simulink model "FM_Stereo_System"  (R2025b)
settings: Solver=FixedStepAuto  StartTime=0.0  StopTime=0.05  FixedStep=Ts  RelTol=1e-3
values from neighbouring files (symbols this model uses):
  Ts = 3e-7    (= 3e-07)    [run_simulink_figures.m]
libraries: dspfdesign x8, commanapbnd3 x2
settings Model: Creator=alfre  LastModifiedBy=alfre

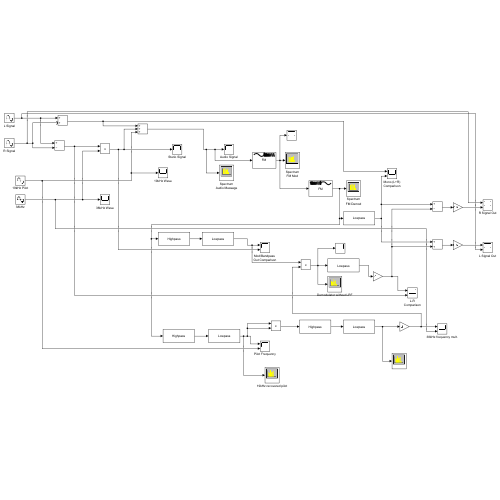
[thumbnail: Simulink's stored preview of the top-level diagram]
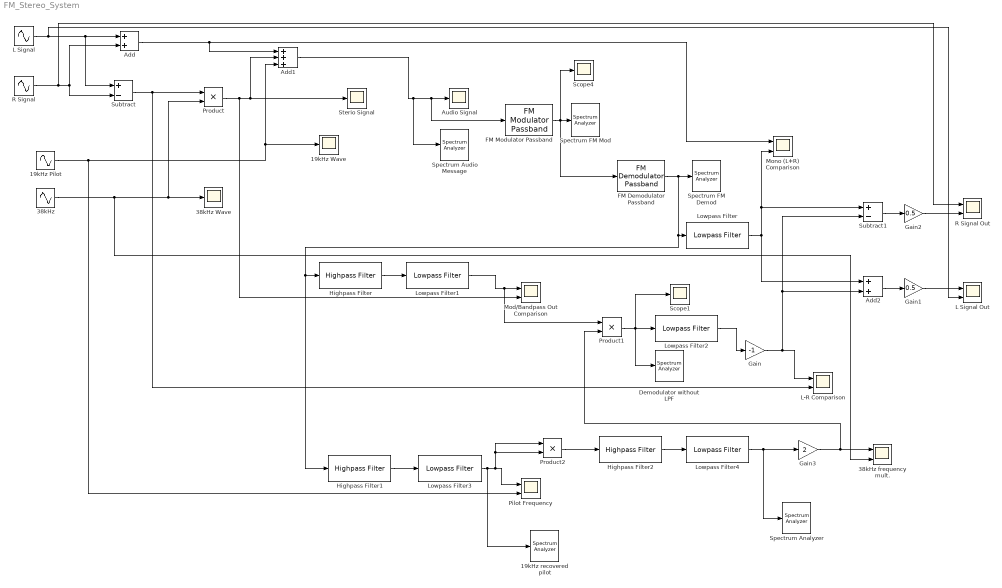
== system FM_Stereo_System ==
  19kHz Pilot : Sin  Frequency=2*pi*19e3  SampleTime=Ts
  19kHz Wave : Scope
      settings: ActiveDisplayYMinimum=-1.1232444431414552  ActiveDisplayYMaximum=1.0699700669461434
  19kHz recovered pilot : SpectrumAnalyzer  WindowPosition=[1.000000,49.000000,1536.000000,793.000000,]  ScopeFrameLocation=window  RBWSource=Property  RBW=100  WindowInvariantSamplesPerUpdate=on  SpectrumUnits=Watts  YLimits=[-0.0301 0.2709]
      settings: OpenAtSimulationStart=off
  38kHz : Sin  Frequency=2*pi*38e3  SampleTime=Ts
  38kHz Wave : Scope
      settings: ActiveDisplayYMinimum=-1.2499013052548038  ActiveDisplayYMaximum=1.2499013052546617  DataLoggingVariableName=ScopeData3
  38kHz frequency mult. : Scope  NumInputPorts=2
      settings: ActiveDisplayYMinimum=-1.6002148562068126  ActiveDisplayYMaximum=1.6003264057017721  DataLoggingVariableName=ScopeData11
  Add : Sum
  Add1 : Sum  Inputs=+++
  Add2 : Sum
  Audio Signal : Scope
      settings: ActiveDisplayYMinimum=-3.9231489006957236  ActiveDisplayYMaximum=3.472021736199153  DataLoggingVariableName=ScopeData2
  Demodulator without LPF : SpectrumAnalyzer  WindowPosition=[1.000000,49.000000,1536.000000,793.000000,]  ScopeFrameLocation=window  RBWSource=Property  RBW=20  WindowInvariantSamplesPerUpdate=on  Span=3333333.3333333335  StartFrequency=-1666666.6666666667  StopFrequency=1666666.6666666667  SpectrumUnits=Watts  YLimits=[-0.0061 0.055]  SelectedToolstripTab=spectrumAnalyzerToolstrip.measurementsTab
      settings: OpenAtSimulationStart=off
  FM Demodulator Passband : commanapbnd3/FM Demodulator Passband  Fc=1e6  Ph=0  Kc=75e3  Ho=100
  FM Modulator Passband : commanapbnd3/FM Modulator Passband  Fc=1e6  Ph=0  Kc=75e3
  Gain : Gain  Gain=-1
  Gain1 : Gain  Gain=0.5
  Gain2 : Gain  Gain=0.5
  Gain3 : Gain  Gain=2
  Highpass Filter : dspfdesign/Highpass Filter  FilterType=IIR  DesignForMinimumOrder=on  FilterOrder=50  StopbandFrequency=20e3  PassbandFrequency=23e3  StopbandAttenuation=80  PassbandRipple=0.1  SampleRate=1e8  SimulateUsing=Interpreted execution  roundingMode=Floor  coeffsDataTypeStr=fixdt(1,16)
  Highpass Filter1 : dspfdesign/Highpass Filter  FilterType=IIR  DesignForMinimumOrder=on  FilterOrder=50  StopbandFrequency=17e3  PassbandFrequency=18.5e3  StopbandAttenuation=80  PassbandRipple=0.1  SampleRate=1e8  SimulateUsing=Interpreted execution  roundingMode=Floor  coeffsDataTypeStr=fixdt(1,16)
  Highpass Filter2 : dspfdesign/Highpass Filter  FilterType=IIR  DesignForMinimumOrder=on  FilterOrder=50  StopbandFrequency=10e3  PassbandFrequency=20e3  StopbandAttenuation=80  PassbandRipple=0.1  SampleRate=44100  SimulateUsing=Interpreted execution  roundingMode=Floor  coeffsDataTypeStr=fixdt(1,16)
  L Signal : Sin  Frequency=2*pi*200  SampleTime=Ts
  L Signal Out : Scope  NumInputPorts=2
      settings: ActiveDisplayYMinimum=-3.4964332783058403  ActiveDisplayYMaximum=3.3980373393108643  DataLoggingVariableName=ScopeData9
  L-R Comparison : Scope  NumInputPorts=2
      settings: ActiveDisplayYMinimum=-2.4471106007113335  ActiveDisplayYMaximum=2.4471106007114405  DataLoggingVariableName=ScopeData7
  Lowpass Filter : dspfdesign/Lowpass Filter  FilterType=IIR  DesignForMinimumOrder=on  FilterOrder=50  PassbandFrequency=15e3  StopbandFrequency=18e3  PassbandRipple=0.1  StopbandAttenuation=80  SampleRate=1e8  SimulateUsing=Interpreted execution  roundingMode=Floor  coeffsDataTypeStr=fixdt(1,16)
  Lowpass Filter1 : dspfdesign/Lowpass Filter  FilterType=IIR  DesignForMinimumOrder=on  FilterOrder=50  PassbandFrequency=50e3  StopbandFrequency=53e3  PassbandRipple=0.1  StopbandAttenuation=80  SampleRate=1e8  SimulateUsing=Interpreted execution  roundingMode=Floor  coeffsDataTypeStr=fixdt(1,16)
  Lowpass Filter2 : dspfdesign/Lowpass Filter  FilterType=IIR  DesignForMinimumOrder=on  FilterOrder=50  PassbandFrequency=15e3  StopbandFrequency=25e3  PassbandRipple=0.1  StopbandAttenuation=80  SampleRate=1e8  SimulateUsing=Interpreted execution  roundingMode=Floor  coeffsDataTypeStr=fixdt(1,16)
  Lowpass Filter3 : dspfdesign/Lowpass Filter  FilterType=IIR  DesignForMinimumOrder=on  FilterOrder=50  PassbandFrequency=19.5e3  StopbandFrequency=21e3  PassbandRipple=0.1  StopbandAttenuation=80  SampleRate=1e8  SimulateUsing=Interpreted execution  roundingMode=Floor  coeffsDataTypeStr=fixdt(1,16)
  Lowpass Filter4 : dspfdesign/Lowpass Filter  FilterType=IIR  DesignForMinimumOrder=on  FilterOrder=50  PassbandFrequency=45e3  StopbandFrequency=55e3  PassbandRipple=0.1  StopbandAttenuation=80  SampleRate=44100  SimulateUsing=Interpreted execution  roundingMode=Floor  coeffsDataTypeStr=fixdt(1,16)
  Mod/Bandpass Out Comparison : Scope  NumInputPorts=2
      settings: ActiveDisplayYMinimum=-1.429366739506019  ActiveDisplayYMaximum=1.5745385313420126  DataLoggingVariableName=ScopeData6
  Mono (L+R) Comparison : Scope  NumInputPorts=2
      settings: ActiveDisplayYMinimum=-2.6609223923967495  ActiveDisplayYMaximum=2.8377619061840487  DataLoggingVariableName=ScopeData5
  Pilot Frequency : Scope  NumInputPorts=2
      settings: ActiveDisplayYMinimum=-1.4181261193129304  ActiveDisplayYMaximum=1.4173969700676226  DataLoggingVariableName=ScopeData10
  Product : Product
  Product1 : Product
  Product2 : Product
  R Signal : Sin  Frequency=2*pi*500  SampleTime=Ts
  R Signal Out : Scope  NumInputPorts=2
      settings: ActiveDisplayYMinimum=-8.3748708297258716  ActiveDisplayYMaximum=8.079178666111769  DataLoggingVariableName=ScopeData8
  Scope1 : Scope
      settings: ActiveDisplayYMinimum=-0.12695669828327838  ActiveDisplayYMaximum=0.10772919385124505  DataLoggingVariableName=ScopeData12
  Scope4 : Scope
      settings: ActiveDisplayYMinimum=-2.0799073223737636  ActiveDisplayYMaximum=1.4385933271441069  DataLoggingVariableName=ScopeData4
  Spectrum Analyzer : SpectrumAnalyzer  WindowPosition=[1.000000,49.000000,1536.000000,793.000000,]  ScopeFrameLocation=window  RBWSource=Property  RBW=100  WindowInvariantSamplesPerUpdate=on  SpectrumUnits=Watts  YLimits=[-0.0074 0.0665]
      settings: OpenAtSimulationStart=off
  Spectrum Audio Message : SpectrumAnalyzer  WindowPosition=[230.000000,227.000000,800.000000,500.000000,]  ScopeFrameLocation=window  RBWSource=Property  RBW=10  WindowInvariantSamplesPerUpdate=on  Span=228000.00000000003  StartFrequency=-114000.00000000001  StopFrequency=114000.00000000001  SpectrumUnits=Watts  YLimits=[-0.0312 0.2812]  SelectedToolstripTab=spectrumAnalyzerToolstrip.measurementsTab
      settings: OpenAtSimulationStart=off
  Spectrum FM Demod : SpectrumAnalyzer  WindowPosition=[1066.000000,234.000000,810.000000,468.000000,]  ScopeFrameLocation=window  SampleRate=44.1e3  PlotAsTwoSidedSpectrum=off  WindowInvariantSamplesPerUpdate=on  FrequencySpan=Start and stop frequencies  StartFrequency=0  StopFrequency=50000  SpectrumUnits=Watts  YLimits=[-0.0211 0.1902]  SelectedToolstripTab=spectrumAnalyzerToolstrip.estimationTab
      settings: OpenAtSimulationStart=off
  Spectrum FM Mod : SpectrumAnalyzer  WindowPosition=[-85.000000,-58.000000,1539.000000,844.000000,]  ScopeFrameLocation=window  SampleRate=44.1e3  PlotAsTwoSidedSpectrum=off  RBWSource=Property  WindowInvariantSamplesPerUpdate=on  FrequencySpan=Start and stop frequencies  StartFrequency=0  StopFrequency=1.5e6  SpectrumUnits=Watts  MaximizeAxes=Off  YLimits=[-0.0000021897 0.000019707]  SelectedToolstripTab=spectrumAnalyzerToolstrip.estimationTab
      settings: OpenAtSimulationStart=off
  Sterio Signal : Scope
      settings: ActiveDisplayYMinimum=-2.353942135145783  ActiveDisplayYMaximum=2.3904316789841289
  Subtract : Sum  Inputs=+-
  Subtract1 : Sum  Inputs=+-
  wires:
  L Signal/1 -> L Signal Out/2, Add/1, Subtract/1
  R Signal/1 -> R Signal Out/1, Subtract/2, Add/2
  Subtract/1 -> L-R Comparison/2, Product/1
  38kHz/1 -> 38kHz frequency mult./2, 38kHz Wave/1, Product/2
  Add/1 -> Mono (L+R) Comparison/1, Add1/1
  Product/1 -> Mod/Bandpass Out Comparison/2, Add1/2, Sterio Signal/1
  19kHz Pilot/1 -> Pilot Frequency/2, 19kHz Wave/1, Add1/3
  Add1/1 -> Spectrum Audio Message/1, FM Modulator Passband/1, Audio Signal/1
  FM Modulator Passband/1 -> FM Demodulator Passband/1, Spectrum FM Mod/1, Scope4/1
  FM Demodulator Passband/1 -> Highpass Filter/1, Highpass Filter1/1, Lowpass Filter/1, Spectrum FM Demod/1
  Lowpass Filter/1 -> Add2/1, Mono (L+R) Comparison/2, Subtract1/1
  Highpass Filter/1 -> Lowpass Filter1/1
  Lowpass Filter1/1 -> Product1/1, Mod/Bandpass Out Comparison/1
  Product1/1 -> Demodulator without LPF/1, Scope1/1, Lowpass Filter2/1
  Lowpass Filter2/1 -> Gain/1
  Add2/1 -> Gain1/1
  Subtract1/1 -> Gain2/1
  Gain1/1 -> L Signal Out/1
  Gain2/1 -> R Signal Out/2
  Highpass Filter1/1 -> Lowpass Filter3/1
  Lowpass Filter3/1 -> 19kHz recovered pilot/1, Product2/2, Product2/1, Pilot Frequency/1
  Product2/1 -> Highpass Filter2/1
  Highpass Filter2/1 -> Lowpass Filter4/1
  Lowpass Filter4/1 -> Spectrum Analyzer/1, Gain3/1
  Gain3/1 -> Product1/2, 38kHz frequency mult./1
  Gain/1 -> Add2/2, Subtract1/2, L-R Comparison/1
